simulink model "powertrain_model"  (R2025a)
settings: Solver=ode23tb  StartTime=0.0  StopTime=simlength  FixedStep=tc  MaxStep=tc
values from neighbouring files (symbols this model uses):
  angle_error = angle_error_deg/180*pi    (= 0)    [init_model.m]
  CTRPIFF_CLIP_RELEASE = 0.001    [init_model.m]
  dead_time = dead_time_INV    (= 4.2e-07)    [init_model.m]
  dead_time_INV = 0.42e-6    (= 4.2e-07)    [init_model.m]
  DThs_init = 0    [init_model.m]
  emf_fb_p = 0.2    [init_model.m]
  emf_fb_p_ccaller_1 = emf_fb_p    (= 0.2)    [init_model.m]
  emf_fb_p_ccaller_2 = emf_fb_p    (= 0.2)    [init_model.m]
  emf_p = emf_fb_p*4/10    (= 0.08)    [init_model.m]
  emf_p_ccaller_1 = emf_fb_p_ccaller_1*4/10    (= 0.08)    [init_model.m]
  emf_p_ccaller_2 = emf_fb_p_ccaller_2*4/10    (= 0.08)    [init_model.m]
  fPWM_INV = 25e3    (= 25000)    [init_model.m]
  g0_reference_flt = fcut_reference_flt * ts_inv * 2*pi    (= 0.00100530964915)    [init_model.m]
  g1_reference_flt = 1 - g0_reference_flt    (= 0.998994690351)    [init_model.m]
  id_ref_if_pu = iload_rms_ref*sqrt(2)/ibez    [init_model.m]
  kalman_omega = kw    [init_model.m]
  kalman_theta = kg    [init_model.m]
  kg = K(1)    [init_model.m]
  ki_id = 2    [analysis_cc.m]    (also in init_model.m = 9)
  ki_iq = 9    [init_model.m]
  ki_w = 1    [init_model.m]
  kp_id = 0.15    [analysis_cc.m]    (also in init_model.m = 0.25)
  kp_iq = 0.2    [init_model.m]
  kp_w = 1    [init_model.m]
  kw = K(2)    [init_model.m]
  luenberger_l1 = Klo(1)    [init_model.m]
  luenberger_l2 = Klo(2)    [init_model.m]
  luenberger_l3 = Klo(3)    [init_model.m]
  motorc_m_scale = 2/3*Vdc_bez/ubez    [init_model.m]
  number_of_cells = 100    [init_model.m]
  omega_flt_fcut = 10    [init_model.m]
  omega_flt_g0 = omega_flt_fcut * ts_inv * 2*pi    (= 0.00251327412287)    [init_model.m]
  omega_flt_g1 = 1 - omega_flt_g0    (= 0.997486725877)    [init_model.m]
  omega_ref_if_pu = 1200*2*pi/omega_bez    [init_model.m]
  phase_compensation_omega = 0    [init_model.m]
  pwm_out_lim = 1    [init_model.m]
  Q = 10    [init_model.m]
  q1Kalman = ts_inv^2    (= 1.6e-09)    [init_model.m]
  q2Kalman = ts_inv^1    (= 4e-05)    [init_model.m]
  q3Kalman = 0    [init_model.m]
  rKalman = 1    [init_model.m]
  Tambient = 1    [init_model.m]
  tc = ts_inv/200    (= 2e-07)    [init_model.m]
  time_init = 0.025    [init_model.m]
  torque_ref = 64/ibez*torque_mode    [init_model.m]
  ts_inv = 1/fPWM_INV    (= 4e-05)    [init_model.m]
  tsample = ts_inv    (= 4e-05)    [init_model.m]
  u_flt_g0 = u_flt_fcut * ts_inv * 2*pi    (= 0.904778684234)    [init_model.m]
  u_flt_g1 = 1 - u_flt_g0    (= 0.0952213157661)    [init_model.m]
  Vdc_bez = 400    [init_model.m]
undefined symbols (not defined in the file or in its folder): b, ibez, Jm, Jm_norm, Ld_norm, Lq_norm, Ls_norm, magnitude, omega_bez, psi_bez, psi_m, psi_m_norm, R_RLload, Rload_eq, Rs_norm, tau_bez, weigth
libraries: fl_lib x100, nesl_utility x84, ee_lib x11, cstblocks x4, lithium_ion_cell_lib x1, simulink x1, pmsm_uvw_with_harmonics_lib x1, pmsm_spatial_harmonics_uvw_lib x1, flexshaft_lib x1
(part 4 of 6)

== system powertrain_model/battery_system/battery_system/LithiumIonBattery/SOC_estimator ==
  Kalman_observer : Subsystem
  SOC*/SOC : Scope  Commented=on  NumInputPorts=2
      settings: SampleTime=tsample  ActiveDisplayYMinimum=-0.16149  ActiveDisplayYMaximum=0.90685
  Selector1 : Selector  InputPortWidth=3  IndexOptions=Index vector (dialog)  Indices=3  OutputSizes=1
  h_hat/h : Scope  Commented=on  NumInputPorts=2
      settings: SampleTime=tsample  ActiveDisplayYMinimum=-0.13002  ActiveDisplayYMaximum=0.15534  DataLoggingVariableName=ScopeData2
  i_out/v_out : Scope  Commented=on  NumInputPorts=2
      settings: SampleTime=tsample  ActiveDisplayYMinimum=-467.64425  ActiveDisplayYMaximum=280.87629  DataLoggingVariableName=ScopeData3
  soc/iout : Scope  Commented=on  NumInputPorts=2
      settings: SampleTime=tsample  ActiveDisplayYMinimum=0.19925  ActiveDisplayYMaximum=0.20008  DataLoggingVariableName=ScopeData4
  wires:
  Kalman_observer/2(SOC) -> SOC*/SOC/2
  Kalman_observer/1(x(k+1|k)) -> Selector1/1
  [im] -> i_out/v_out/1  "im+noise"
  [h] -> h_hat/h/2
  [SOC] -> soc/iout/1, SOC*/SOC/1
  Selector1/1 -> h_hat/h/1  "h_hat(z)"
  [vout] -> Kalman_observer/1(vout(k)), i_out/v_out/2
  [icell] -> soc/iout/2

== system powertrain_model/battery_system/battery_system/LithiumIonBattery/lithium ion cell analytical ocv ==
  Current Sensor : fl_lib/Electrical/Electrical Sensors/Current Sensor
  Electrical Reference : fl_lib/Electrical/Electrical Elements/Electrical Reference
  PS Constant : fl_lib/Physical Signals/Sources/PS Constant  constant=298.15 K
  PS-Simulink Converter{,1..4} (5 alike) : nesl_utility/PS-Simulink Converter  PhysicalDomain=network_engine_domain  SubClassName=ps_output  LeftPortType=input  RightPortType=output  PseudoPeriodic=off  Frequencies=[]  VectorFormat=1-D array  Unit=inherit  AffineConversion=off
  Voltage Sensor : fl_lib/Electrical/Electrical Sensors/Voltage Sensor
  lithium-ion battery with analytical OCV : lithium_ion_cell_lib/lithium-ion Cell with analytical OCV  Qcell=Q hr*A  N=number_of_cells  E_1=E1 V  E0=E0 V  E1=E1 V  E2=E2 V  E3=E3 V  Elog=Elog V  R0=R0 Ohm  R1=R1 Ohm  C1=C1 F  M=M V  alpha=alpha  u_specify=off  u_priority=High  u=Vdc V  u_nominal_specify=off  u_nominal_unit=V  u_nominal_value=1  u_ocv_specify=off  u_ocv_priority=High  u_ocv=Vdc V  u_ocv_nominal_specify=off  u_ocv_nominal_unit=V  u_ocv_nominal_value=1  icell_specify=off  icell_priority=None  icell=0 A  icell_nominal_specify=off  icell_nominal_unit=A  icell_nominal_value=1  i_r1_specify=off  i_r1_priority=None  i_r1=0 A  i_r1_nominal_specify=off  i_r1_nominal_unit=A  i_r1_nominal_value=1  z_specify=on  z_priority=High  z=soc_init  z_nominal_specify=off  z_nominal_unit=1  z_nominal_value=1  h_specify=off  h_priority=High  h=0  h_nominal_specify=off  h_nominal_unit=1  h_nominal_value=1
      settings: InternalSimscapePortConfiguration="{\"Bottom\":[],\"Left\":[{\"id\":\"T\",\"label\":\"T\",\"type\":\"input\"}],\"Right\":[{\"id\":\"u_p\",\"label\":\"u+\",\"type\":\"foundation.electrical.electrical\"},{\"id\":\"u_n\",\"label\":\"u-\",\"type\":\"foundation.electrical.electrical\"},{\"id\":\"z_out\",\"label\":\"SOC\",\"type\":\"output\"},{\"id\":\"i_r1_out\",\"label\":\"i_r1\",\"type\":\"output\"},{\"id\":\"h_out\",\"label\":\"hysteresis\",\"type\":\"output\"}],\"Top\":[]}"
  white_noise : Subsystem
  U+ : PMIOPort  Side=Right
  U- : PMIOPort  Port=2  Side=Right
  tag scope: SOC=global, h=global, icell=global, im=global, vout=global
  wires:
  PS-Simulink Converter/1 -> [vout]  "vout(k)"
  PS-Simulink Converter1/1 -> white_noise/1(in)  "i(k)"
  white_noise/1(out) -> [im]
  PS-Simulink Converter4/1 -> [h]  "h(t)"
  PS-Simulink Converter2/1 -> [icell]  "icell"
  PS-Simulink Converter3/1 -> [SOC]  "SOC*"
  connections:
  lithium-ion battery with analytical OCV/LConn1 -- PS Constant/RConn1
  PS-Simulink Converter/LConn1 -- Voltage Sensor/RConn1
  Current Sensor/RConn2 -- Voltage Sensor/LConn1 -- U+/RConn1
  Electrical Reference/LConn1 -- Voltage Sensor/RConn2 -- U-/RConn1 -- lithium-ion battery with analytical OCV/RConn2
  Current Sensor/RConn1 -- PS-Simulink Converter1/LConn1
  lithium-ion battery with analytical OCV/RConn1 -- Current Sensor/LConn1
  lithium-ion battery with analytical OCV/RConn3 -- PS-Simulink Converter3/LConn1
  lithium-ion battery with analytical OCV/RConn4 -- PS-Simulink Converter2/LConn1
  lithium-ion battery with analytical OCV/RConn5 -- PS-Simulink Converter4/LConn1

== system powertrain_model/driver control/bemf_observer/bemf_observer_ccaller/Reset Trigger ==
  Step : Step  Time=time_init  Before=1  After=0  SampleTime=0
  Out1 : Outport
  wires:
  Step/1 -> Out1/1  "Reset"

== system powertrain_model/driver control/bemf_observer/bemf_observer_simulink/double_integrator_observer ==
  theta : Inport
  Gain : Gain  Gain=kw
  Gain1 : Gain  Gain=kg
  Gain2 : Gain  Gain=omega_bez
  Gain3 : Gain  Gain=1/omega_bez
  Gain5 : Gain  Gain=ts_inv
  Sum : Sum  Inputs=-+|
  Sum1 : Sum  Inputs=|++
  Sum2 : Sum  Inputs=|++
  Sum8 : Sum  Inputs=++|
  Unit Delay1 : UnitDelay  SampleTime=ts_inv  HasFrameUpgradeWarning=on
  Unit Delay2 : UnitDelay  SampleTime=ts_inv  HasFrameUpgradeWarning=on
  bounder1 : MATLAB Function  TreatAsAtomicUnit=on  SystemSampleTime=ts_inv
  bounder2 : MATLAB Function  TreatAsAtomicUnit=on  SystemSampleTime=ts_inv
  omega_pu_hat : Outport  VectorParamsAs1DForOutWhenUnconnected=off
  theta_hat : Outport  Port=2  VectorParamsAs1DForOutWhenUnconnected=off
  wires:
  Unit Delay1/1 -> Sum/1, theta_hat/1, Sum2/2  "theta_hat"
  Sum/1 -> bounder1/1(u)
  Gain5/1 -> Gain2/1
  Gain3/1 -> Sum1/1
  Gain2/1 -> Sum8/1
  bounder1/1(y) -> Gain1/1, Gain/1
  bounder2/1(y) -> Unit Delay1/1
  Sum2/1 -> Sum8/2
  Unit Delay2/1 -> Gain5/1, Sum1/2, omega_pu_hat/1
  Gain/1 -> Gain3/1
  Sum1/1 -> Unit Delay2/1
  Sum8/1 -> bounder2/1(u)
  theta/1 -> Sum/2  "theta_bemf"
  Gain1/1 -> Sum2/1

== system powertrain_model/driver control/bemf_observer/bemf_observer_simulink/omega_hat_flt ==
  omega_hat : Inport
  Gain3 : Gain  Gain=omega_flt_g1
  Gain6 : Gain  Gain=omega_flt_g0
  Sum : Sum  Inputs=|++
  Unit Delay1 : UnitDelay  SampleTime=ts_inv  HasFrameUpgradeWarning=on
  omega_hat_flt : Outport  VectorParamsAs1DForOutWhenUnconnected=off
  wires:
  Sum/1 -> omega_hat_flt/1, Unit Delay1/1
  Gain3/1 -> Sum/2
  Unit Delay1/1 -> Gain3/1
  omega_hat/1 -> Gain6/1
  Gain6/1 -> Sum/1

== system powertrain_model/driver control/bemf_observer/bemf_observer_simulink/psi_alpha_hat ==
  ualpha : Inport
  ialpha : Inport  Port=2
  Gain1 : Gain  Gain=Rs_norm
  Gain2 : Gain  Gain=emf_fb_p
  Gain3 : Gain  Gain=emf_p
  Gain4 : Gain  Gain=omega_bez
  Gain5 : Gain  Gain=Ls_norm
  Gain6 : Gain  Gain=motorc_m_scale
  Gain7 : Gain  Gain=ts_inv
  Product : Product  RndMeth=Zero
  Sum : Sum  Inputs=|+-
  Sum1 : Sum  Inputs=|+-
  Sum2 : Sum  Inputs=++-  SaturateOnIntegerOverflow=on
  Sum3 : Sum  Inputs=|++
  Sum4 : Sum  Inputs=+-  SaturateOnIntegerOverflow=on
  Unit Delay1 : UnitDelay  SampleTime=ts_inv  HasFrameUpgradeWarning=on
  psi_s_alpha_hat : Outport  VectorParamsAs1DForOutWhenUnconnected=off
  psi_r_alpha_hat : Outport  Port=2  VectorParamsAs1DForOutWhenUnconnected=off
  wires:
  Gain5/1 -> Sum4/2
  Gain6/1 -> Sum/1
  Product/1 -> Gain6/1
  Gain7/1 -> Sum3/1
  [vdc_pu] -> Product/2
  Gain2/1 -> Sum2/1
  Sum1/1 -> Gain2/1
  Sum3/1 -> Unit Delay1/1  "psi_s_alpha_hat_hat"
  Unit Delay1/1 -> psi_s_alpha_hat/1, Sum4/1, Sum3/2, Gain3/1
  ualpha/1 -> Product/1
  Sum/1 -> Sum2/2
  Gain1/1 -> Sum/2
  ialpha/1 -> Gain1/1, Gain5/1
  Gain3/1 -> Sum2/3
  Sum2/1 -> Gain4/1
  Gain4/1 -> Gain7/1
  [psi_r_alpha_hat] -> Sum1/2
  [psi_r_m_alpha] -> Sum1/1
  Sum4/1 -> psi_r_alpha_hat/1

== system powertrain_model/driver control/bemf_observer/bemf_observer_simulink/psi_beta_hat ==
  ubeta : Inport
  ibeta : Inport  Port=2
  Gain1 : Gain  Gain=Rs_norm
  Gain2 : Gain  Gain=emf_fb_p
  Gain3 : Gain  Gain=emf_p
  Gain4 : Gain  Gain=omega_bez
  Gain5 : Gain  Gain=Ls_norm
  Gain6 : Gain  Gain=motorc_m_scale
  Gain7 : Gain  Gain=ts_inv
  Product : Product  RndMeth=Zero
  Sum : Sum  Inputs=|+-
  Sum1 : Sum  Inputs=|+-
  Sum2 : Sum  Inputs=++-  SaturateOnIntegerOverflow=on
  Sum3 : Sum  Inputs=|++
  Sum4 : Sum  Inputs=+-  SaturateOnIntegerOverflow=on
  Unit Delay1 : UnitDelay  SampleTime=ts_inv  HasFrameUpgradeWarning=on
  psi_s_beta_hat : Outport  VectorParamsAs1DForOutWhenUnconnected=off
  psi_r_beta_hat : Outport  Port=2  VectorParamsAs1DForOutWhenUnconnected=off
  wires:
  Gain5/1 -> Sum4/2
  Gain6/1 -> Sum/1
  Product/1 -> Gain6/1
  Gain7/1 -> Sum3/1
  [vdc_pu] -> Product/2
  ubeta/1 -> Product/1
  Gain2/1 -> Sum2/1
  Sum3/1 -> Unit Delay1/1
  Unit Delay1/1 -> psi_s_beta_hat/1, Sum4/1, Sum3/2, Gain3/1
  [psi_r_m_beta] -> Sum1/1
  [psi_r_beta_hat] -> Sum1/2
  Sum1/1 -> Gain2/1
  Gain4/1 -> Gain7/1
  Sum2/1 -> Gain4/1
  Gain3/1 -> Sum2/3
  ibeta/1 -> Gain1/1, Gain5/1
  Gain1/1 -> Sum/2
  Sum/1 -> Sum2/2
  Sum4/1 -> psi_r_beta_hat/1

== system powertrain_model/driver control/bemf_observer/bemf_observer_simulink/theta_bemf_hat ==
  psi_r_alpha_hat : Inport
  psi_r_beta_hat : Inport  Port=2
  omega_pu_hat : Inport  Port=3
  Sum : Sum  Inputs=|++
  Trigonometric Function : Trigonometry  Operator=atan2  OutputSignalType=real
  phase_compensation_omega : Gain  Gain=phase_compensation_omega
  theta_emf_hat : Outport  VectorParamsAs1DForOutWhenUnconnected=off
  wires:
  Sum/1 -> theta_emf_hat/1
  phase_compensation_omega/1 -> Sum/2
  omega_pu_hat/1 -> phase_compensation_omega/1
  Trigonometric Function/1 -> Sum/1
  psi_r_beta_hat/1 -> Trigonometric Function/1
  psi_r_alpha_hat/1 -> Trigonometric Function/2

== system powertrain_model/driver control/bemf_observer/bemf_observer_with_load_estimator_ccaller/Reset Trigger ==
  Step : Step  Time=time_init  Before=1  After=0  SampleTime=0
  Out1 : Outport
  wires:
  Step/1 -> Out1/1  "Reset"

== system powertrain_model/driver control/current_ctrl/vector_current_ctrl/MTPA ==
  iq_ref : Inport
  id_ref_ext : Inport  Port=2
  Constant : Constant  Value=psi_m_norm
  Gain1 : Gain  Gain=1/(Ld_norm - Lq_norm)/2
  Gain2 : Gain  Gain=1/(Ld_norm - Lq_norm)/2
  Gain3 : Gain  Gain=0
  Math Function1 : Math  Operator=magnitude^2  SignedPower=on
  Math Function4 : Math  Operator=magnitude^2  SignedPower=on
  Sqrt : Sqrt
  Sum : Sum  Inputs=|++
  Sum1 : Sum  Inputs=|--
  Sum3 : Sum  Inputs=|++
  id_ref_pu < x < 0 : Saturate  UpperLimit=0  LowerLimit=-0.15
  id_ref : Outport  VectorParamsAs1DForOutWhenUnconnected=off
  wires:
  Sum1/1 -> id_ref_pu < x < 0/1
  id_ref_pu < x < 0/1 -> Gain3/1
  Math Function4/1 -> Sum/1
  Math Function1/1 -> Sum/2
  Gain1/1 -> Math Function4/1
  Sum/1 -> Sqrt/1
  Sqrt/1 -> Sum1/2
  iq_ref/1 -> Math Function1/1
  Gain2/1 -> Sum1/1
  Constant/1 -> Gain1/1, Gain2/1
  Gain3/1 -> Sum3/1
  Sum3/1 -> id_ref/1
  id_ref_ext/1 -> Sum3/2

== system powertrain_model/driver control/current_ctrl/vector_current_ctrl/dq_vector_pi ==
  id : Inport
  id_ref : Inport  Port=2
  iq : Inport  Port=3
  iq_ref : Inport  Port=4
  Sum1 : Sum  Inputs=|+-
  Sum2 : Sum  Inputs=|+-
  bounder1 : Subsystem
  bounder2 : Subsystem
  pi_d : Subsystem
  pi_q : Subsystem
  switch : Subsystem
  vector lenght : Subsystem
  ctrl_d_u : Outport
  ctrl_q_u : Outport  Port=2
  wires:
  bounder2/2(clip) -> switch/2(clip 2)
  bounder2/1(mq_sat) -> ctrl_q_u/1
  pi_q/1(Vqs_out) -> bounder2/3(mq), vector lenght/2(mq)
  vector lenght/1(m_1) -> bounder1/2(m_1), bounder2/2(m_1)
  vector lenght/2(m) -> bounder1/3(m), bounder2/1(m)
  pi_d/1(ud_out) -> vector lenght/1(md), bounder1/1(md)
  switch/1(clip) -> pi_q/2(clip), pi_d/2(clip)
  bounder1/2(clip) -> switch/1(clip 1)
  Sum2/1 -> pi_q/1(iq_tilde)
  Sum1/1 -> pi_d/1(id_tilde)
  bounder1/1(md_sat) -> ctrl_d_u/1
  id_ref/1 -> Sum1/1
  id/1 -> Sum1/2
  iq_ref/1 -> Sum2/1
  iq/1 -> Sum2/2

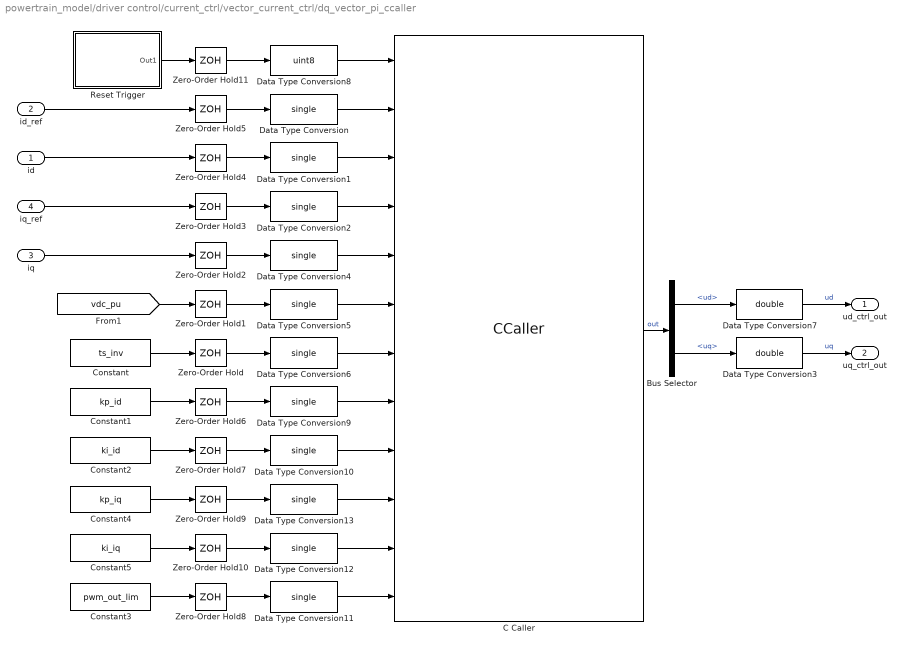
== system powertrain_model/driver control/current_ctrl/vector_current_ctrl/dq_vector_pi_ccaller ==
  id : Inport
  id_ref : Inport  Port=2
  iq : Inport  Port=3
  iq_ref : Inport  Port=4
  Bus Selector : BusSelector  OutputSignals=ud,uq
  C Caller : CCaller  FunctionName=dqvector_pi_process_simulink  PortSpecificationStruct="%)30     .    ,!8   8    (     @         %    \"     T    !     0         %  0 \"0    $    _    07)G3F%M90  4&]R=$YA;64 4V-O<&4     26YD97@     5'EP90      4VEZ90      27-';&]B86P   X    P    !@    @    $          4    (     0    ,    !         !   P!O=70 #@   #     &    \"     0         !0    @    !     P    $         $  # &]U=  .    .     8    (    !          %    \"     $    &     0         0   ...(+7280 chars)"  SampleTime=ts_inv
  Constant : Constant  Value=ts_inv
  Constant1 : Constant  Value=kp_id
  Constant2 : Constant  Value=ki_id
  Constant3 : Constant  Value=pwm_out_lim
  Constant4 : Constant  Value=kp_iq
  Constant5 : Constant  Value=ki_iq
  Data Type Conversion{,1..2,4..6,9..13} (11 alike) : DataTypeConversion  OutDataTypeStr=single  SaturateOnIntegerOverflow=off  RndMeth=Floor
  Data Type Conversion3 : DataTypeConversion  OutDataTypeStr=double  SaturateOnIntegerOverflow=off  RndMeth=Floor
  Data Type Conversion7 : DataTypeConversion  OutDataTypeStr=double  SaturateOnIntegerOverflow=off  RndMeth=Floor
  Data Type Conversion8 : DataTypeConversion  OutDataTypeStr=uint8  SaturateOnIntegerOverflow=off  RndMeth=Floor
  Reset Trigger : Subsystem
  Zero-Order Hold{,1..11} (12 alike) : ZeroOrderHold  SampleTime=ts_inv
  ud_ctrl_out : Outport
  uq_ctrl_out : Outport  Port=2
  wires:
  Data Type Conversion5/1 -> C Caller/6
  Data Type Conversion/1 -> C Caller/2
  Data Type Conversion1/1 -> C Caller/3
  Data Type Conversion4/1 -> C Caller/5
  Data Type Conversion2/1 -> C Caller/4
  Data Type Conversion6/1 -> C Caller/7
  Zero-Order Hold/1 -> Data Type Conversion6/1
  Zero-Order Hold5/1 -> Data Type Conversion/1
  Zero-Order Hold4/1 -> Data Type Conversion1/1
  Zero-Order Hold3/1 -> Data Type Conversion2/1
  Zero-Order Hold2/1 -> Data Type Conversion4/1
  Zero-Order Hold1/1 -> Data Type Conversion5/1
  [vdc_pu] -> Zero-Order Hold1/1
  Constant/1 -> Zero-Order Hold/1
  id_ref/1 -> Zero-Order Hold5/1
  iq_ref/1 -> Zero-Order Hold3/1
  id/1 -> Zero-Order Hold4/1
  iq/1 -> Zero-Order Hold2/1
  Data Type Conversion7/1 -> ud_ctrl_out/1  "ud"
  Data Type Conversion3/1 -> uq_ctrl_out/1  "uq"
  Reset Trigger/1(Out1) -> Zero-Order Hold11/1
  Data Type Conversion8/1 -> C Caller/1
  Constant1/1 -> Zero-Order Hold6/1
  Zero-Order Hold6/1 -> Data Type Conversion9/1
  Data Type Conversion9/1 -> C Caller/8
  Data Type Conversion10/1 -> C Caller/9
  Zero-Order Hold7/1 -> Data Type Conversion10/1
  Zero-Order Hold8/1 -> Data Type Conversion11/1
  Constant2/1 -> Zero-Order Hold7/1
  Constant3/1 -> Zero-Order Hold8/1
  Data Type Conversion11/1 -> C Caller/12
  Constant5/1 -> Zero-Order Hold10/1
  Zero-Order Hold10/1 -> Data Type Conversion12/1
  Zero-Order Hold9/1 -> Data Type Conversion13/1
  Constant4/1 -> Zero-Order Hold9/1
  Data Type Conversion13/1 -> C Caller/10
  Data Type Conversion12/1 -> C Caller/11
  C Caller/1 -> Bus Selector/1  "out"
  Bus Selector/1 -> Data Type Conversion7/1  "<ud>"
  Bus Selector/2 -> Data Type Conversion3/1  "<uq>"
  Zero-Order Hold11/1 -> Data Type Conversion8/1

== system powertrain_model/inverter/MOS based inverter/inverter/inverter_mosfet_leg_thermal ==
  Simulink-PS Converter{,1..5} (6 alike) : nesl_utility/Simulink-PS Converter  PhysicalDomain=network_engine_domain  SubClassName=ps_input  LeftPortType=input  RightPortType=output  PseudoPeriodic=off  Frequencies=[]  NoiseDistribution=none  NoiseParameters=[]  Unit=V  AffineConversion=on  FilteringAndDerivatives=provide  SimscapeFilterOrder=1  InputFilterTimeConstant=0.001  UdotUserProvided=0
  mosfet_3 : Subsystem
      settings: PortSchema="{\"entries\":[{\"content\":{\"sides\":[{\"content\":{\"connectorIds\":[\"LConn1\"]},\"type\":\"ConnectorPlacement.EquallySpacedRectSide\",\"uuid\":\"9277da8d-d460-43e6-8478-dd662f15d226\"},{\"content\":{\"connectorIds\":[],\"side\":\"RIGHT\"},\"type\":\"ConnectorPlacement.EquallySpacedRectSide\",\"uuid\":\"a7ece396-f1d9-4f4f-a05b-db1fc65d6e1d\"},{\"content\":{\"connectorIds\":[\"LConn2\"],\"side\":\"TOP\"},\"type\":\"ConnectorPlacement.EquallySpacedRectSide\",\"uuid\":\"fdd70777-e9cf-4317-afb6-cae87f75d5b0\"},{\"content\":{\"connectorIds\":[\"RConn1\"],\"side\":\"BOTTOM\"},\"type\":\"ConnectorPlacement.EquallySpacedRectSide\",\"uuid\":\"2353ed68-b1a1-4775-9ca9-31e268d5443b\"}]},\"type\":\"ConnectorPlacement.EquallySpacedConnector\",\"uuid\":\"d5479f4c-4e65-4791-adcb-73df11f88590\"}],\"packageUris\":[\"http://schema.mathworks.com/mf0/Connector/R2020b\"],\"version\":\"1.0\"}"
  mosfet_4 : Subsystem
      settings: PortSchema="{\"entries\":[{\"content\":{\"sides\":[{\"content\":{\"connectorIds\":[\"LConn1\"]},\"type\":\"ConnectorPlacement.EquallySpacedRectSide\",\"uuid\":\"9277da8d-d460-43e6-8478-dd662f15d226\"},{\"content\":{\"connectorIds\":[],\"side\":\"RIGHT\"},\"type\":\"ConnectorPlacement.EquallySpacedRectSide\",\"uuid\":\"a7ece396-f1d9-4f4f-a05b-db1fc65d6e1d\"},{\"content\":{\"connectorIds\":[\"LConn2\"],\"side\":\"TOP\"},\"type\":\"ConnectorPlacement.EquallySpacedRectSide\",\"uuid\":\"fdd70777-e9cf-4317-afb6-cae87f75d5b0\"},{\"content\":{\"connectorIds\":[\"RConn1\"],\"side\":\"BOTTOM\"},\"type\":\"ConnectorPlacement.EquallySpacedRectSide\",\"uuid\":\"2353ed68-b1a1-4775-9ca9-31e268d5443b\"}]},\"type\":\"ConnectorPlacement.EquallySpacedConnector\",\"uuid\":\"d5479f4c-4e65-4791-adcb-73df11f88590\"}],\"packageUris\":[\"http://schema.mathworks.com/mf0/Connector/R2020b\"],\"version\":\"1.0\"}"
  mosfet_5 : Subsystem
      settings: PortSchema="{\"entries\":[{\"content\":{\"sides\":[{\"content\":{\"connectorIds\":[\"LConn1\"]},\"type\":\"ConnectorPlacement.EquallySpacedRectSide\",\"uuid\":\"9277da8d-d460-43e6-8478-dd662f15d226\"},{\"content\":{\"connectorIds\":[],\"side\":\"RIGHT\"},\"type\":\"ConnectorPlacement.EquallySpacedRectSide\",\"uuid\":\"a7ece396-f1d9-4f4f-a05b-db1fc65d6e1d\"},{\"content\":{\"connectorIds\":[\"LConn2\"],\"side\":\"TOP\"},\"type\":\"ConnectorPlacement.EquallySpacedRectSide\",\"uuid\":\"fdd70777-e9cf-4317-afb6-cae87f75d5b0\"},{\"content\":{\"connectorIds\":[\"RConn1\"],\"side\":\"BOTTOM\"},\"type\":\"ConnectorPlacement.EquallySpacedRectSide\",\"uuid\":\"2353ed68-b1a1-4775-9ca9-31e268d5443b\"}]},\"type\":\"ConnectorPlacement.EquallySpacedConnector\",\"uuid\":\"d5479f4c-4e65-4791-adcb-73df11f88590\"}],\"packageUris\":[\"http://schema.mathworks.com/mf0/Connector/R2020b\"],\"version\":\"1.0\"}"
  mosfet_6 : Subsystem
      settings: PortSchema="{\"entries\":[{\"content\":{\"sides\":[{\"content\":{\"connectorIds\":[\"LConn1\"]},\"type\":\"ConnectorPlacement.EquallySpacedRectSide\",\"uuid\":\"9277da8d-d460-43e6-8478-dd662f15d226\"},{\"content\":{\"connectorIds\":[],\"side\":\"RIGHT\"},\"type\":\"ConnectorPlacement.EquallySpacedRectSide\",\"uuid\":\"a7ece396-f1d9-4f4f-a05b-db1fc65d6e1d\"},{\"content\":{\"connectorIds\":[\"LConn2\"],\"side\":\"TOP\"},\"type\":\"ConnectorPlacement.EquallySpacedRectSide\",\"uuid\":\"fdd70777-e9cf-4317-afb6-cae87f75d5b0\"},{\"content\":{\"connectorIds\":[\"RConn1\"],\"side\":\"BOTTOM\"},\"type\":\"ConnectorPlacement.EquallySpacedRectSide\",\"uuid\":\"2353ed68-b1a1-4775-9ca9-31e268d5443b\"}]},\"type\":\"ConnectorPlacement.EquallySpacedConnector\",\"uuid\":\"d5479f4c-4e65-4791-adcb-73df11f88590\"}],\"packageUris\":[\"http://schema.mathworks.com/mf0/Connector/R2020b\"],\"version\":\"1.0\"}"
  mosfet_thermal_1 : Subsystem
      settings: PortSchema="{\"entries\":[{\"content\":{\"sides\":[{\"content\":{\"connectorIds\":[\"LConn1\"]},\"type\":\"ConnectorPlacement.EquallySpacedRectSide\",\"uuid\":\"9277da8d-d460-43e6-8478-dd662f15d226\"},{\"content\":{\"connectorIds\":[],\"side\":\"RIGHT\"},\"type\":\"ConnectorPlacement.EquallySpacedRectSide\",\"uuid\":\"a7ece396-f1d9-4f4f-a05b-db1fc65d6e1d\"},{\"content\":{\"connectorIds\":[\"LConn2\"],\"side\":\"TOP\"},\"type\":\"ConnectorPlacement.EquallySpacedRectSide\",\"uuid\":\"fdd70777-e9cf-4317-afb6-cae87f75d5b0\"},{\"content\":{\"connectorIds\":[\"RConn1\"],\"side\":\"BOTTOM\"},\"type\":\"ConnectorPlacement.EquallySpacedRectSide\",\"uuid\":\"2353ed68-b1a1-4775-9ca9-31e268d5443b\"}]},\"type\":\"ConnectorPlacement.EquallySpacedConnector\",\"uuid\":\"d5479f4c-4e65-4791-adcb-73df11f88590\"}],\"packageUris\":[\"http://schema.mathworks.com/mf0/Connector/R2020b\"],\"version\":\"1.0\"}"
  mosfet_thermal_2 : Subsystem
      settings: PortSchema="{\"entries\":[{\"content\":{\"sides\":[{\"content\":{\"connectorIds\":[\"LConn1\"]},\"type\":\"ConnectorPlacement.EquallySpacedRectSide\",\"uuid\":\"9277da8d-d460-43e6-8478-dd662f15d226\"},{\"content\":{\"connectorIds\":[],\"side\":\"RIGHT\"},\"type\":\"ConnectorPlacement.EquallySpacedRectSide\",\"uuid\":\"a7ece396-f1d9-4f4f-a05b-db1fc65d6e1d\"},{\"content\":{\"connectorIds\":[\"LConn2\"],\"side\":\"TOP\"},\"type\":\"ConnectorPlacement.EquallySpacedRectSide\",\"uuid\":\"fdd70777-e9cf-4317-afb6-cae87f75d5b0\"},{\"content\":{\"connectorIds\":[\"RConn1\"],\"side\":\"BOTTOM\"},\"type\":\"ConnectorPlacement.EquallySpacedRectSide\",\"uuid\":\"2353ed68-b1a1-4775-9ca9-31e268d5443b\"}]},\"type\":\"ConnectorPlacement.EquallySpacedConnector\",\"uuid\":\"d5479f4c-4e65-4791-adcb-73df11f88590\"}],\"packageUris\":[\"http://schema.mathworks.com/mf0/Connector/R2020b\"],\"version\":\"1.0\"}"
  udc(+) : PMIOPort  Side=Left
  u : PMIOPort  Port=2  Side=Right
  v : PMIOPort  Port=3  Side=Right
  w : PMIOPort  Port=4  Side=Right
  udc(-) : PMIOPort  Port=5  Side=Left
  wires:
  [gm2] -> Simulink-PS Converter1/1
  [gm3] -> Simulink-PS Converter2/1
  [gm4] -> Simulink-PS Converter3/1
  [gm5] -> Simulink-PS Converter4/1
  [gm1] -> Simulink-PS Converter/1
  [gm6] -> Simulink-PS Converter5/1
  connections:
  mosfet_thermal_2/LConn1 -- Simulink-PS Converter1/RConn1
  mosfet_thermal_2/RConn1 -- udc(-)/RConn1 -- mosfet_6/RConn1 -- mosfet_4/RConn1
  mosfet_6/LConn2 -- w/RConn1 -- mosfet_5/RConn1
  mosfet_5/LConn1 -- Simulink-PS Converter4/RConn1
  mosfet_4/LConn2 -- v/RConn1 -- mosfet_3/RConn1
  Simulink-PS Converter/RConn1 -- mosfet_thermal_1/LConn1
  mosfet_4/LConn1 -- Simulink-PS Converter3/RConn1
  mosfet_thermal_1/RConn1 -- u/RConn1 -- mosfet_thermal_2/LConn2
  mosfet_thermal_1/LConn2 -- udc(+)/RConn1 -- mosfet_5/LConn2 -- mosfet_3/LConn2
  mosfet_6/LConn1 -- Simulink-PS Converter5/RConn1
  mosfet_3/LConn1 -- Simulink-PS Converter2/RConn1

== system powertrain_model/inverter/MOS based inverter/inverter/inverter_without_mosfet_leg_thermal ==
  Simulink-PS Converter{,1..5} (6 alike) : nesl_utility/Simulink-PS Converter  PhysicalDomain=network_engine_domain  SubClassName=ps_input  LeftPortType=input  RightPortType=output  PseudoPeriodic=off  Frequencies=[]  NoiseDistribution=none  NoiseParameters=[]  Unit=V  AffineConversion=on  FilteringAndDerivatives=provide  SimscapeFilterOrder=1  InputFilterTimeConstant=0.001  UdotUserProvided=0
  mosfet_1 : Subsystem
      settings: PortSchema="{\"entries\":[{\"content\":{\"sides\":[{\"content\":{\"connectorIds\":[\"LConn1\"]},\"type\":\"ConnectorPlacement.EquallySpacedRectSide\",\"uuid\":\"9277da8d-d460-43e6-8478-dd662f15d226\"},{\"content\":{\"connectorIds\":[],\"side\":\"RIGHT\"},\"type\":\"ConnectorPlacement.EquallySpacedRectSide\",\"uuid\":\"a7ece396-f1d9-4f4f-a05b-db1fc65d6e1d\"},{\"content\":{\"connectorIds\":[\"LConn2\"],\"side\":\"TOP\"},\"type\":\"ConnectorPlacement.EquallySpacedRectSide\",\"uuid\":\"fdd70777-e9cf-4317-afb6-cae87f75d5b0\"},{\"content\":{\"connectorIds\":[\"RConn1\"],\"side\":\"BOTTOM\"},\"type\":\"ConnectorPlacement.EquallySpacedRectSide\",\"uuid\":\"2353ed68-b1a1-4775-9ca9-31e268d5443b\"}]},\"type\":\"ConnectorPlacement.EquallySpacedConnector\",\"uuid\":\"d5479f4c-4e65-4791-adcb-73df11f88590\"}],\"packageUris\":[\"http://schema.mathworks.com/mf0/Connector/R2020b\"],\"version\":\"1.0\"}"
  mosfet_2 : Subsystem
      settings: PortSchema="{\"entries\":[{\"content\":{\"sides\":[{\"content\":{\"connectorIds\":[\"LConn1\"]},\"type\":\"ConnectorPlacement.EquallySpacedRectSide\",\"uuid\":\"9277da8d-d460-43e6-8478-dd662f15d226\"},{\"content\":{\"connectorIds\":[],\"side\":\"RIGHT\"},\"type\":\"ConnectorPlacement.EquallySpacedRectSide\",\"uuid\":\"a7ece396-f1d9-4f4f-a05b-db1fc65d6e1d\"},{\"content\":{\"connectorIds\":[\"LConn2\"],\"side\":\"TOP\"},\"type\":\"ConnectorPlacement.EquallySpacedRectSide\",\"uuid\":\"fdd70777-e9cf-4317-afb6-cae87f75d5b0\"},{\"content\":{\"connectorIds\":[\"RConn1\"],\"side\":\"BOTTOM\"},\"type\":\"ConnectorPlacement.EquallySpacedRectSide\",\"uuid\":\"2353ed68-b1a1-4775-9ca9-31e268d5443b\"}]},\"type\":\"ConnectorPlacement.EquallySpacedConnector\",\"uuid\":\"d5479f4c-4e65-4791-adcb-73df11f88590\"}],\"packageUris\":[\"http://schema.mathworks.com/mf0/Connector/R2020b\"],\"version\":\"1.0\"}"
  mosfet_3 : Subsystem
      settings: PortSchema="{\"entries\":[{\"content\":{\"sides\":[{\"content\":{\"connectorIds\":[\"LConn1\"]},\"type\":\"ConnectorPlacement.EquallySpacedRectSide\",\"uuid\":\"9277da8d-d460-43e6-8478-dd662f15d226\"},{\"content\":{\"connectorIds\":[],\"side\":\"RIGHT\"},\"type\":\"ConnectorPlacement.EquallySpacedRectSide\",\"uuid\":\"a7ece396-f1d9-4f4f-a05b-db1fc65d6e1d\"},{\"content\":{\"connectorIds\":[\"LConn2\"],\"side\":\"TOP\"},\"type\":\"ConnectorPlacement.EquallySpacedRectSide\",\"uuid\":\"fdd70777-e9cf-4317-afb6-cae87f75d5b0\"},{\"content\":{\"connectorIds\":[\"RConn1\"],\"side\":\"BOTTOM\"},\"type\":\"ConnectorPlacement.EquallySpacedRectSide\",\"uuid\":\"2353ed68-b1a1-4775-9ca9-31e268d5443b\"}]},\"type\":\"ConnectorPlacement.EquallySpacedConnector\",\"uuid\":\"d5479f4c-4e65-4791-adcb-73df11f88590\"}],\"packageUris\":[\"http://schema.mathworks.com/mf0/Connector/R2020b\"],\"version\":\"1.0\"}"
  mosfet_4 : Subsystem
      settings: PortSchema="{\"entries\":[{\"content\":{\"sides\":[{\"content\":{\"connectorIds\":[\"LConn1\"]},\"type\":\"ConnectorPlacement.EquallySpacedRectSide\",\"uuid\":\"9277da8d-d460-43e6-8478-dd662f15d226\"},{\"content\":{\"connectorIds\":[],\"side\":\"RIGHT\"},\"type\":\"ConnectorPlacement.EquallySpacedRectSide\",\"uuid\":\"a7ece396-f1d9-4f4f-a05b-db1fc65d6e1d\"},{\"content\":{\"connectorIds\":[\"LConn2\"],\"side\":\"TOP\"},\"type\":\"ConnectorPlacement.EquallySpacedRectSide\",\"uuid\":\"fdd70777-e9cf-4317-afb6-cae87f75d5b0\"},{\"content\":{\"connectorIds\":[\"RConn1\"],\"side\":\"BOTTOM\"},\"type\":\"ConnectorPlacement.EquallySpacedRectSide\",\"uuid\":\"2353ed68-b1a1-4775-9ca9-31e268d5443b\"}]},\"type\":\"ConnectorPlacement.EquallySpacedConnector\",\"uuid\":\"d5479f4c-4e65-4791-adcb-73df11f88590\"}],\"packageUris\":[\"http://schema.mathworks.com/mf0/Connector/R2020b\"],\"version\":\"1.0\"}"
  mosfet_5 : Subsystem
      settings: PortSchema="{\"entries\":[{\"content\":{\"sides\":[{\"content\":{\"connectorIds\":[\"LConn1\"]},\"type\":\"ConnectorPlacement.EquallySpacedRectSide\",\"uuid\":\"9277da8d-d460-43e6-8478-dd662f15d226\"},{\"content\":{\"connectorIds\":[],\"side\":\"RIGHT\"},\"type\":\"ConnectorPlacement.EquallySpacedRectSide\",\"uuid\":\"a7ece396-f1d9-4f4f-a05b-db1fc65d6e1d\"},{\"content\":{\"connectorIds\":[\"LConn2\"],\"side\":\"TOP\"},\"type\":\"ConnectorPlacement.EquallySpacedRectSide\",\"uuid\":\"fdd70777-e9cf-4317-afb6-cae87f75d5b0\"},{\"content\":{\"connectorIds\":[\"RConn1\"],\"side\":\"BOTTOM\"},\"type\":\"ConnectorPlacement.EquallySpacedRectSide\",\"uuid\":\"2353ed68-b1a1-4775-9ca9-31e268d5443b\"}]},\"type\":\"ConnectorPlacement.EquallySpacedConnector\",\"uuid\":\"d5479f4c-4e65-4791-adcb-73df11f88590\"}],\"packageUris\":[\"http://schema.mathworks.com/mf0/Connector/R2020b\"],\"version\":\"1.0\"}"
  mosfet_6 : Subsystem
      settings: PortSchema="{\"entries\":[{\"content\":{\"sides\":[{\"content\":{\"connectorIds\":[\"LConn1\"]},\"type\":\"ConnectorPlacement.EquallySpacedRectSide\",\"uuid\":\"9277da8d-d460-43e6-8478-dd662f15d226\"},{\"content\":{\"connectorIds\":[],\"side\":\"RIGHT\"},\"type\":\"ConnectorPlacement.EquallySpacedRectSide\",\"uuid\":\"a7ece396-f1d9-4f4f-a05b-db1fc65d6e1d\"},{\"content\":{\"connectorIds\":[\"LConn2\"],\"side\":\"TOP\"},\"type\":\"ConnectorPlacement.EquallySpacedRectSide\",\"uuid\":\"fdd70777-e9cf-4317-afb6-cae87f75d5b0\"},{\"content\":{\"connectorIds\":[\"RConn1\"],\"side\":\"BOTTOM\"},\"type\":\"ConnectorPlacement.EquallySpacedRectSide\",\"uuid\":\"2353ed68-b1a1-4775-9ca9-31e268d5443b\"}]},\"type\":\"ConnectorPlacement.EquallySpacedConnector\",\"uuid\":\"d5479f4c-4e65-4791-adcb-73df11f88590\"}],\"packageUris\":[\"http://schema.mathworks.com/mf0/Connector/R2020b\"],\"version\":\"1.0\"}"
  udc(+) : PMIOPort  Side=Left
  u : PMIOPort  Port=2  Side=Right
  v : PMIOPort  Port=3  Side=Right
  w : PMIOPort  Port=4  Side=Right
  udc(-) : PMIOPort  Port=5  Side=Left
  wires:
  [gm6] -> Simulink-PS Converter5/1
  [gm1] -> Simulink-PS Converter/1
  [gm5] -> Simulink-PS Converter4/1
  [gm4] -> Simulink-PS Converter3/1
  [gm3] -> Simulink-PS Converter2/1
  [gm2] -> Simulink-PS Converter1/1
  connections:
  mosfet_3/LConn1 -- Simulink-PS Converter2/RConn1
  mosfet_6/LConn1 -- Simulink-PS Converter5/RConn1
  udc(+)/RConn1 -- mosfet_1/LConn2 -- mosfet_3/LConn2 -- mosfet_5/LConn2
  u/RConn1 -- mosfet_2/LConn2 -- mosfet_1/RConn1
  mosfet_4/LConn1 -- Simulink-PS Converter3/RConn1
  mosfet_1/LConn1 -- Simulink-PS Converter/RConn1
  v/RConn1 -- mosfet_3/RConn1 -- mosfet_4/LConn2
  mosfet_5/LConn1 -- Simulink-PS Converter4/RConn1
  w/RConn1 -- mosfet_5/RConn1 -- mosfet_6/LConn2
  udc(-)/RConn1 -- mosfet_2/RConn1 -- mosfet_4/RConn1 -- mosfet_6/RConn1
  mosfet_2/LConn1 -- Simulink-PS Converter1/RConn1

== system powertrain_model/inverter/MOS based inverter/sv_pwm/modulator ==
  u : Inport
  v : Inport  Port=2
  w : Inport  Port=3
  Bus Creator : BusCreator  Inputs=2
  Bus Creator1 : BusCreator  Inputs=2
  Bus Creator2 : BusCreator  Inputs=2
  Bus Creator3 : BusCreator  Inputs=3
  Gain{,1..5} (6 alike) : Gain  Gain=15
  PWM generator 1 : Subsystem  mask{f=fPWM_INV, ph=0, m_up=1, m_low=0, dead_time=dead_time_INV}
      mask prompts: f "Frequency"; ph "Phase"; m_up "Max Input Modulation Value"; m_low "Min Input Modulation Value"; dead_time "Dead Time"
  PWM generator 2 : Subsystem  mask{f=fPWM_INV, ph=0, m_up=1, m_low=0, dead_time=dead_time_INV}
      mask prompts: f "Frequency"; ph "Phase"; m_up "Max Input Modulation Value"; m_low "Min Input Modulation Value"; dead_time "Dead Time"
  PWM generator 3 : Subsystem  mask{f=fPWM_INV, ph=0, m_up=1, m_low=0, dead_time=dead_time_INV}
      mask prompts: f "Frequency"; ph "Phase"; m_up "Max Input Modulation Value"; m_low "Min Input Modulation Value"; dead_time "Dead Time"
  firing_gates : Outport
  wires:
  u/1 -> PWM generator 1/1(m_index)
  w/1 -> PWM generator 3/1(m_index)
  v/1 -> PWM generator 2/1(m_index)
  Bus Creator3/1 -> firing_gates/1
  Bus Creator1/1 -> Bus Creator3/2
  Bus Creator2/1 -> Bus Creator3/3
  PWM generator 1/1(m1) -> Gain/1
  PWM generator 1/2(m2) -> Gain1/1
  PWM generator 2/1(m1) -> Gain2/1
  PWM generator 2/2(m2) -> Gain3/1
  PWM generator 3/1(m1) -> Gain4/1
  PWM generator 3/2(m2) -> Gain5/1
  Gain/1 -> Bus Creator/1
  Gain1/1 -> Bus Creator/2
  Gain2/1 -> Bus Creator1/1
  Gain3/1 -> Bus Creator1/2
  Gain4/1 -> Bus Creator2/1
  Gain5/1 -> Bus Creator2/2
  Bus Creator/1 -> Bus Creator3/1

== system powertrain_model/inverter/MOS based inverter/sv_pwm/modulator1 ==
  u : Inport
  v : Inport  Port=2
  w : Inport  Port=3
  Bus Creator : BusCreator  Inputs=2
  Bus Creator1 : BusCreator  Inputs=2
  Bus Creator2 : BusCreator  Inputs=2
  Bus Creator3 : BusCreator  Inputs=3
  Gain{,1..5} (6 alike) : Gain  Gain=15
  PWM generator 1 : Subsystem  mask{f=fPWM_INV, ph=0, m_up=1, m_low=0, dead_time=0}
      mask prompts: f "Frequency"; ph "Phase"; m_up "Max Input Modulation Value"; m_low "Min Input Modulation Value"; dead_time "Dead Time"
  PWM generator 2 : Subsystem  mask{f=fPWM_INV, ph=0, m_up=1, m_low=0, dead_time=0}
      mask prompts: f "Frequency"; ph "Phase"; m_up "Max Input Modulation Value"; m_low "Min Input Modulation Value"; dead_time "Dead Time"
  PWM generator 3 : Subsystem  mask{f=fPWM_INV, ph=0, m_up=1, m_low=0, dead_time=0}
      mask prompts: f "Frequency"; ph "Phase"; m_up "Max Input Modulation Value"; m_low "Min Input Modulation Value"; dead_time "Dead Time"
  firing_gates : Outport
  wires:
  Bus Creator/1 -> Bus Creator3/1
  Gain5/1 -> Bus Creator2/2
  Gain4/1 -> Bus Creator2/1
  Gain3/1 -> Bus Creator1/2
  Gain2/1 -> Bus Creator1/1
  Gain1/1 -> Bus Creator/2
  Gain/1 -> Bus Creator/1
  PWM generator 3/2(m2) -> Gain5/1
  PWM generator 3/1(m1) -> Gain4/1
  PWM generator 2/2(m2) -> Gain3/1
  PWM generator 2/1(m1) -> Gain2/1
  PWM generator 1/2(m2) -> Gain1/1
  PWM generator 1/1(m1) -> Gain/1
  Bus Creator2/1 -> Bus Creator3/3
  Bus Creator1/1 -> Bus Creator3/2
  Bus Creator3/1 -> firing_gates/1
  v/1 -> PWM generator 2/1(m_index)
  w/1 -> PWM generator 3/1(m_index)
  u/1 -> PWM generator 1/1(m_index)

== system powertrain_model/inverter/MOS based inverter/threePhsModulator/PWM generator 1 ==
  m_index : Inport
  Constant : Constant  Value=dead_time*f*2
  Data Type Conversion1 : DataTypeConversion
  Data Type Conversion2 : DataTypeConversion
  Gain : Gain  Gain=1/(pi/2)
  Gain2 : Gain  Gain=gate_voltage
  Gain3 : Gain  Gain=gate_voltage
  Hit Crossing : HitCross  ShowOutputPort=off
  Hit Crossing1 : HitCross  ShowOutputPort=off
  Relational Operator1 : RelationalOperator  Operator=<=  InputSameDT=off
  Relational Operator2 : RelationalOperator  Operator=<=  InputSameDT=off
  Saturation1 : Saturate  UpperLimit=m_up  LowerLimit=m_low
  Sine Wave : Sin  Frequency=f*2*pi  Phase=-pi/2+ph  SampleTime=0
  Sum : Sum  Inputs=|++  SaturateOnIntegerOverflow=on
  Sum1 : Sum  Inputs=-+|  SaturateOnIntegerOverflow=on
  Trigonometric Function1 : Trigonometry  Operator=asin
  m1 : Outport
  m2 : Outport  Port=2
  wires:
  Relational Operator1/1 -> Data Type Conversion1/1
  m_index/1 -> Saturation1/1
  Data Type Conversion1/1 -> Gain2/1, Hit Crossing/1
  Relational Operator2/1 -> Data Type Conversion2/1
  Data Type Conversion2/1 -> Gain3/1, Hit Crossing1/1
  Constant/1 -> Sum/2, Sum1/1
  Saturation1/1 -> Sum/1, Sum1/2
  Sum/1 -> Relational Operator1/1
  Sum1/1 -> Relational Operator2/2
  Sine Wave/1 -> Trigonometric Function1/1
  Trigonometric Function1/1 -> Gain/1
  Gain/1 -> Relational Operator1/2, Relational Operator2/1
  Gain2/1 -> m1/1
  Gain3/1 -> m2/1

== system powertrain_model/inverter/MOS based inverter/threePhsModulator/PWM generator 2 ==
  m_index : Inport
  Constant : Constant  Value=dead_time*f*2
  Data Type Conversion1 : DataTypeConversion
  Data Type Conversion2 : DataTypeConversion
  Gain : Gain  Gain=1/(pi/2)
  Gain2 : Gain  Gain=gate_voltage
  Gain3 : Gain  Gain=gate_voltage
  Hit Crossing : HitCross  ShowOutputPort=off
  Hit Crossing1 : HitCross  ShowOutputPort=off
  Relational Operator1 : RelationalOperator  Operator=<=  InputSameDT=off
  Relational Operator2 : RelationalOperator  Operator=<=  InputSameDT=off
  Saturation1 : Saturate  UpperLimit=m_up  LowerLimit=m_low
  Sine Wave : Sin  Frequency=f*2*pi  Phase=-pi/2+ph  SampleTime=0
  Sum : Sum  Inputs=|++  SaturateOnIntegerOverflow=on
  Sum1 : Sum  Inputs=-+|  SaturateOnIntegerOverflow=on
  Trigonometric Function1 : Trigonometry  Operator=asin
  m1 : Outport
  m2 : Outport  Port=2
  wires:
  Gain3/1 -> m2/1
  Gain2/1 -> m1/1
  Gain/1 -> Relational Operator2/1, Relational Operator1/2
  Trigonometric Function1/1 -> Gain/1
  Sine Wave/1 -> Trigonometric Function1/1
  Sum1/1 -> Relational Operator2/2
  Sum/1 -> Relational Operator1/1
  Saturation1/1 -> Sum1/2, Sum/1
  Constant/1 -> Sum1/1, Sum/2
  Data Type Conversion2/1 -> Hit Crossing1/1, Gain3/1
  Relational Operator2/1 -> Data Type Conversion2/1
  Data Type Conversion1/1 -> Hit Crossing/1, Gain2/1
  m_index/1 -> Saturation1/1
  Relational Operator1/1 -> Data Type Conversion1/1

== system powertrain_model/inverter/MOS based inverter/threePhsModulator/PWM generator 3 ==
  m_index : Inport
  Constant : Constant  Value=dead_time*f*2
  Data Type Conversion1 : DataTypeConversion
  Data Type Conversion2 : DataTypeConversion
  Gain : Gain  Gain=1/(pi/2)
  Gain2 : Gain  Gain=gate_voltage
  Gain3 : Gain  Gain=gate_voltage
  Hit Crossing : HitCross  ShowOutputPort=off
  Hit Crossing1 : HitCross  ShowOutputPort=off
  Relational Operator1 : RelationalOperator  Operator=<=  InputSameDT=off
  Relational Operator2 : RelationalOperator  Operator=<=  InputSameDT=off
  Saturation1 : Saturate  UpperLimit=m_up  LowerLimit=m_low
  Sine Wave : Sin  Frequency=f*2*pi  Phase=-pi/2+ph  SampleTime=0
  Sum : Sum  Inputs=|++  SaturateOnIntegerOverflow=on
  Sum1 : Sum  Inputs=-+|  SaturateOnIntegerOverflow=on
  Trigonometric Function1 : Trigonometry  Operator=asin
  m1 : Outport
  m2 : Outport  Port=2
  wires:
  Relational Operator1/1 -> Data Type Conversion1/1
  m_index/1 -> Saturation1/1
  Data Type Conversion1/1 -> Gain2/1, Hit Crossing/1
  Relational Operator2/1 -> Data Type Conversion2/1
  Data Type Conversion2/1 -> Gain3/1, Hit Crossing1/1
  Constant/1 -> Sum/2, Sum1/1
  Saturation1/1 -> Sum/1, Sum1/2
  Sum/1 -> Relational Operator1/1
  Sum1/1 -> Relational Operator2/2
  Sine Wave/1 -> Trigonometric Function1/1
  Trigonometric Function1/1 -> Gain/1
  Gain/1 -> Relational Operator1/2, Relational Operator2/1
  Gain2/1 -> m1/1
  Gain3/1 -> m2/1

== system powertrain_model/inverter/MOS based inverter/threePhsModulator/Third harmonic injecting ==
  m1 : Inport
  m2 : Inport  Port=2
  m3 : Inport  Port=3
  Gain : Gain  Gain=1/2
  MinMax : MinMax  Function=max  Inputs=3
  MinMax1 : MinMax  Inputs=3
  Sum : Sum  Inputs=|++
  thind_H : Outport
  wires:
  m2/1 -> MinMax/2, MinMax1/2
  m1/1 -> MinMax/1, MinMax1/1
  m3/1 -> MinMax/3, MinMax1/3
  MinMax/1 -> Sum/1
  MinMax1/1 -> Sum/2
  Sum/1 -> Gain/1
  Gain/1 -> thind_H/1

== system powertrain_model/battery_system/battery_system/LithiumIonBattery/SOC_estimator/Kalman_observer ==
  vout(k) : Inport
  Constant : Constant  Value=tsample
  Constant1 : Constant  Value=Q
  Constant2 : Constant  Value=q1Kalman
  Constant3 : Constant  Value=q2Kalman
  Constant4 : Constant  Value=q3Kalman
  Constant5 : Constant  Value=rKalman
  Constant6 : Constant  Value=tsample
  Constant7 : Constant  Value=Q
  Selector : Selector  InputPortWidth=3  IndexOptions=Index vector (dialog)  Indices=1  OutputSizes=1
  Unit Delay4 : UnitDelay  SampleTime=tsample  HasFrameUpgradeWarning=on
  kalman_observer_gains : MATLAB Function  TreatAsAtomicUnit=on  SystemSampleTime=tsample
  lithium-ion battery model : MATLAB Function  TreatAsAtomicUnit=on  SystemSampleTime=tsample
  vout/vout_hat : Scope  Commented=on  NumInputPorts=2
      settings: SampleTime=tsample  ActiveDisplayYMinimum=-781.71351  ActiveDisplayYMaximum=896.62262
  x(k+1|k) : Outport
  SOC : Outport  Port=2
  wires:
  lithium-ion battery model/2(u) -> vout/vout_hat/2  "vout_hat"
  vout(k)/1 -> lithium-ion battery model/7(vout), vout/vout_hat/1
  lithium-ion battery model/3(x) -> x(k+1|k)/1, Selector/1  "x(k+1|k)"
  kalman_observer_gains/2(l2) -> lithium-ion battery model/5(l2)
  Constant6/1 -> kalman_observer_gains/2(ts)
  lithium-ion battery model/1(SOC) -> SOC/1  "SOC"
  Constant7/1 -> kalman_observer_gains/8(Q)
  kalman_observer_gains/3(l3) -> lithium-ion battery model/6(l3)
  Constant1/1 -> lithium-ion battery model/3(Q)
  Constant5/1 -> kalman_observer_gains/7(r)
  [im] -> kalman_observer_gains/1(i)
  Constant4/1 -> kalman_observer_gains/6(q3)
  Constant2/1 -> kalman_observer_gains/4(q1)
  kalman_observer_gains/1(l1) -> lithium-ion battery model/4(l1)
  Constant/1 -> lithium-ion battery model/2(ts)
  Constant3/1 -> kalman_observer_gains/5(q2)
  Unit Delay4/1 -> kalman_observer_gains/3(z)  "x(k|k-1)"
  Selector/1 -> Unit Delay4/1
  [im] -> lithium-ion battery model/1(i)
